simulink model "gnc_PathServer"  (R2026b)
settings: Solver=VariableStepAuto
values from neighbouring files (symbols this model uses):
  Ts = prm.Ts    [gnc_missionFSM.m]    (also in gnc_mpcPlantUpdate.m)
undefined symbols (not defined in the file or in its folder): P
libraries: drivinglib x3, simulink x2
settings Model: Creator=aomar  LastModifiedBy=aomar

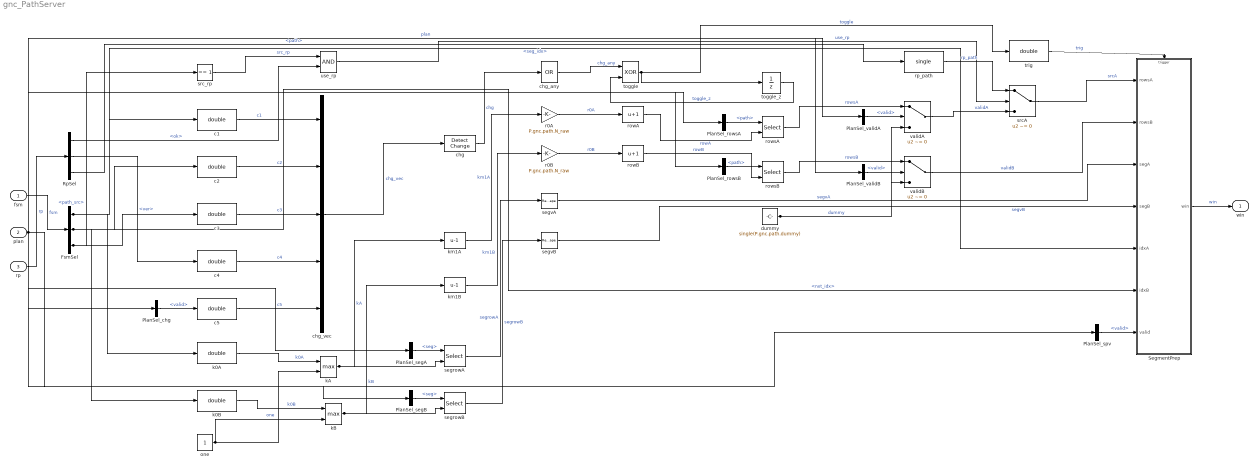
== system gnc_PathServer ==
  fsm : Inport  OutDataTypeStr=Bus: Bus_FsmOut  SampleTime=Ts.gnc
  plan : Inport  Port=2  OutDataTypeStr=Bus: Bus_MissionPlan
  rp : Inport  Port=3  OutDataTypeStr=Bus: Bus_ReplanResult  SampleTime=Ts.gnc
  FsmSel : BusSelector  OutputSignals=seg_idx,nxt_idx,path_src
  PlanSel_chg : BusSelector  OutputSignals=valid
  PlanSel_rowsA : BusSelector  OutputSignals=path
  PlanSel_rowsB : BusSelector  OutputSignals=path
  PlanSel_segA : BusSelector  OutputSignals=seg
  PlanSel_segB : BusSelector  OutputSignals=seg
  PlanSel_spv : BusSelector  OutputSignals=valid
  PlanSel_validA : BusSelector  OutputSignals=valid
  PlanSel_validB : BusSelector  OutputSignals=valid
  RpSel : BusSelector  OutputSignals=ok,ver,path
  SegmentPrep : Subsystem  TreatAsAtomicUnit=on
  c{1..5} (5 alike) : DataTypeConversion  OutDataTypeStr=double  RndMeth=Nearest
  chg : simulink/Logic and Bit Operations/Detect Change  vinit=0  OutDataTypeStr=boolean
  chg_any : Logic  Operator=OR  Inputs=1  AllPortsSameDT=off  OutDataTypeStr=boolean
  chg_vec : Concatenate  NumInputs=5
  dummy : Constant  Value=single(P.gnc.path.dummy)  OutDataTypeStr=single
  k0A : DataTypeConversion  OutDataTypeStr=double  RndMeth=Nearest
  k0B : DataTypeConversion  OutDataTypeStr=double  RndMeth=Nearest
  kA : MinMax  Function=max  Inputs=2
  kB : MinMax  Function=max  Inputs=2
  km1A : Bias  Bias=-1  SaturateOnIntegerOverflow=off
  km1B : Bias  Bias=-1  SaturateOnIntegerOverflow=off
  one : Constant  OutDataTypeStr=double  SampleTime=Ts.gnc
  r0A : Gain  Gain=P.gnc.path.N_raw
  r0B : Gain  Gain=P.gnc.path.N_raw
  rowA : Bias  Bias=1  SaturateOnIntegerOverflow=off
  rowB : Bias  Bias=1  SaturateOnIntegerOverflow=off
  rowsA : Selector  NumberOfDimensions=2  InputPortWidth=3  IndexOptions=Starting index (port),Select all  Indices=,  OutputSizes=P.gnc.path.N_raw,1
  rowsB : Selector  NumberOfDimensions=2  InputPortWidth=3  IndexOptions=Starting index (port),Select all  Indices=,  OutputSizes=P.gnc.path.N_raw,1
  rp_path : DataTypeConversion  OutDataTypeStr=single  RndMeth=Nearest
  segrowA : Selector  NumberOfDimensions=2  InputPortWidth=3  IndexOptions=Index vector (port),Select all  Indices=,  OutputSizes=1
  segrowB : Selector  NumberOfDimensions=2  InputPortWidth=3  IndexOptions=Index vector (port),Select all  Indices=,  OutputSizes=1
  segvA : Reshape
  segvB : Reshape
  srcA : Switch  Criteria=u2 ~= 0  SaturateOnIntegerOverflow=off  InputSameDT=off
  src_rp : simulink/Logic and Bit Operations/Compare To Constant  relop===  const=1  OutDataTypeStr=boolean
  toggle : Logic  Operator=XOR  AllPortsSameDT=off  OutDataTypeStr=boolean
  toggle_z : UnitDelay  InitialCondition=false  SampleTime=Ts.gnc
  trig : DataTypeConversion  OutDataTypeStr=double  RndMeth=Nearest
  use_rp : Logic  AllPortsSameDT=off  OutDataTypeStr=boolean
  validA : Switch  Criteria=u2 ~= 0  SaturateOnIntegerOverflow=off  InputSameDT=off
  validB : Switch  Criteria=u2 ~= 0  SaturateOnIntegerOverflow=off  InputSameDT=off
  win : Outport  OutDataTypeStr=Bus: Bus_PathWindow
  wires:
  fsm/1 -> FsmSel/1  "fsm"
  plan/1 -> PlanSel_segB/1, PlanSel_segA/1, PlanSel_validA/1, PlanSel_rowsA/1, PlanSel_spv/1, PlanSel_chg/1, PlanSel_rowsB/1, PlanSel_validB/1  "plan"
  rp/1 -> RpSel/1  "rp"
  RpSel/1 -> use_rp/2  "<ok>"
  RpSel/2 -> c4/1  "<ver>"
  RpSel/3 -> rp_path/1  "<path>"
  FsmSel/1 -> k0A/1, c1/1, SegmentPrep/5(idxA)  "<seg_idx>"
  FsmSel/2 -> k0B/1, c2/1, SegmentPrep/6(idxB)  "<nxt_idx>"
  FsmSel/3 -> src_rp/1, c3/1  "<path_src>"
  PlanSel_chg/1 -> c5/1  "<valid>"
  src_rp/1 -> use_rp/1  "src_rp"
  one/1 -> kA/2, kB/2  "one"
  c1/1 -> chg_vec/1  "c1"
  c2/1 -> chg_vec/2  "c2"
  c3/1 -> chg_vec/3  "c3"
  c4/1 -> chg_vec/4  "c4"
  c5/1 -> chg_vec/5  "c5"
  k0A/1 -> kA/1  "k0A"
  k0B/1 -> kB/1  "k0B"
  chg_vec/1 -> chg/1  "chg_vec"
  use_rp/1 -> srcA/2  "use_rp"
  kA/1 -> km1A/1, segrowA/2  "kA"
  kB/1 -> km1B/1, segrowB/2  "kB"
  PlanSel_segA/1 -> segrowA/1  "<seg>"
  PlanSel_segB/1 -> segrowB/1  "<seg>"
  km1A/1 -> r0A/1  "km1A"
  km1B/1 -> r0B/1  "km1B"
  segrowA/1 -> segvA/1  "segrowA"
  segrowB/1 -> segvB/1  "segrowB"
  chg/1 -> chg_any/1  "chg"
  chg_any/1 -> toggle/1  "chg_any"
  r0A/1 -> rowA/1  "r0A"
  r0B/1 -> rowB/1  "r0B"
  segvA/1 -> SegmentPrep/3(segA)  "segvA"
  segvB/1 -> SegmentPrep/4(segB)  "segvB"
  toggle/1 -> trig/1, toggle_z/1  "toggle"
  rowA/1 -> rowsA/2  "rowA"
  rowB/1 -> rowsB/2  "rowB"
  PlanSel_rowsA/1 -> rowsA/1  "<path>"
  PlanSel_rowsB/1 -> rowsB/1  "<path>"
  dummy/1 -> validA/3, validB/3  "dummy"
  toggle_z/1 -> toggle/2  "toggle_z"
  rowsA/1 -> validA/1  "rowsA"
  rowsB/1 -> validB/1  "rowsB"
  PlanSel_validA/1 -> validA/2  "<valid>"
  PlanSel_validB/1 -> validB/2  "<valid>"
  validA/1 -> srcA/3  "validA"
  validB/1 -> SegmentPrep/2(rowsB)  "validB"
  rp_path/1 -> srcA/1  "rp_path"
  srcA/1 -> SegmentPrep/1(rowsA)  "srcA"
  trig/1 -> SegmentPrep/Trigger  "trig"
  PlanSel_spv/1 -> SegmentPrep/7(valid)  "<valid>"
  SegmentPrep/1(win) -> win/1  "win"

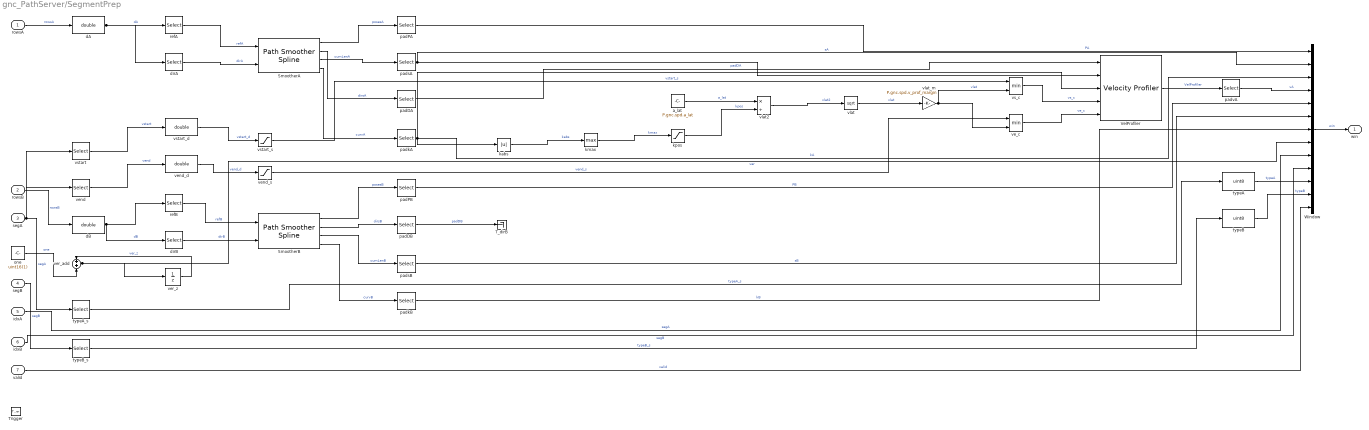
== system gnc_PathServer/SegmentPrep ==
  rowsA : Inport
  rowsB : Inport  Port=2
  segA : Inport  Port=3
  segB : Inport  Port=4
  idxA : Inport  Port=5
  idxB : Inport  Port=6
  valid : Inport  Port=7
  Trigger : TriggerPort  TriggerType=either  VariantControl=(inherit)  InitialTriggerSignalState=zero  PortDimensions=1
  SmootherA : drivinglib/Path Smoother Spline  NumSmoothPoses=P.gnc.path.N_smooth  MinSeparation=1e-3  SampleTime=-1  ShowOptionalOutports=on  SimulateUsing=Code generation
  SmootherB : drivinglib/Path Smoother Spline  NumSmoothPoses=P.gnc.path.N_smooth  MinSeparation=1e-3  SampleTime=-1  ShowOptionalOutports=on  SimulateUsing=Code generation
  T_dirB : Terminator
  VelProfiler : drivinglib/Velocity Profiler  MaxLongitudinalAccel=P.gnc.spd.a_acc  MaxLongitudinalDecel=P.gnc.spd.a_dec  MaxSpeed=P.gnc.spd.v_max  MaxLongitudinalJerk=P.gnc.spd.jerk  MaxLateralAccel=P.gnc.spd.a_lat  ShowOptionalOutport=off  SampleTime=-1  SimulateUsing=Code generation
  Window : BusCreator  Inputs=13  OutDataTypeStr=Bus: Bus_PathWindow  NonVirtualBus=on
  a_lat : Constant  Value=P.gnc.spd.a_lat  OutDataTypeStr=double  SampleTime=-1
  dA : DataTypeConversion  OutDataTypeStr=double  RndMeth=Nearest
  dB : DataTypeConversion  OutDataTypeStr=double  RndMeth=Nearest
  dirA : Selector  NumberOfDimensions=2  InputPortWidth=3  IndexOptions=Select all,Index vector (dialog)  Indices=,4  OutputSizes=1
  dirB : Selector  NumberOfDimensions=2  InputPortWidth=3  IndexOptions=Select all,Index vector (dialog)  Indices=,4  OutputSizes=1
  kabs : Abs  SaturateOnIntegerOverflow=off
  kmax : MinMax  Function=max
  kpos : Saturate  UpperLimit=inf  LowerLimit=1e-9
  one : Constant  Value=uint16(1)  OutDataTypeStr=uint16  SampleTime=-1
  padDA : Selector  IndexOptions=Index vector (dialog)  Indices=1:P.gnc.path.N_smooth  OutputSizes=1
  padDB : Selector  IndexOptions=Index vector (dialog)  Indices=1:P.gnc.path.N_smooth  OutputSizes=1
  padPA : Selector  NumberOfDimensions=2  InputPortWidth=3  IndexOptions=Index vector (dialog),Index vector (dialog)  Indices=1:P.gnc.path.N_smooth,[1 2 3]  OutputSizes=1
  padPB : Selector  NumberOfDimensions=2  InputPortWidth=3  IndexOptions=Index vector (dialog),Index vector (dialog)  Indices=1:P.gnc.path.N_smooth,[1 2 3]  OutputSizes=1
  padkA : Selector  IndexOptions=Index vector (dialog)  Indices=1:P.gnc.path.N_smooth  OutputSizes=1
  padkB : Selector  IndexOptions=Index vector (dialog)  Indices=1:P.gnc.path.N_smooth  OutputSizes=1
  padsA : Selector  IndexOptions=Index vector (dialog)  Indices=1:P.gnc.path.N_smooth  OutputSizes=1
  padsB : Selector  IndexOptions=Index vector (dialog)  Indices=1:P.gnc.path.N_smooth  OutputSizes=1
  padvA : Selector  IndexOptions=Index vector (dialog)  Indices=1:P.gnc.path.N_smooth  OutputSizes=1
  refA : Selector  NumberOfDimensions=2  InputPortWidth=3  IndexOptions=Select all,Index vector (dialog)  Indices=,[1 2 3]  OutputSizes=1
  refB : Selector  NumberOfDimensions=2  InputPortWidth=3  IndexOptions=Select all,Index vector (dialog)  Indices=,[1 2 3]  OutputSizes=1
  typeA : DataTypeConversion  OutDataTypeStr=uint8  RndMeth=Nearest
  typeA_s : Selector  IndexOptions=Index vector (dialog)  Indices=1  OutputSizes=1
  typeB : DataTypeConversion  OutDataTypeStr=uint8  RndMeth=Nearest
  typeB_s : Selector  IndexOptions=Index vector (dialog)  Indices=1  OutputSizes=1
  ve_c : MinMax  Inputs=2
  vend : Selector  IndexOptions=Index vector (dialog)  Indices=5  OutputSizes=1
  vend_d : DataTypeConversion  OutDataTypeStr=double  RndMeth=Nearest
  vend_s : Saturate  UpperLimit=P.gnc.spd.v_max  LowerLimit=0
  ver_add : Sum  OutDataTypeStr=uint16
  ver_z : UnitDelay  InitialCondition=uint16(0)  SampleTime=-1
  vlat : Sqrt
  vlat2 : Product  Inputs=*/
  vlat_m : Gain  Gain=P.gnc.spd.v_prof_margin
  vs_c : MinMax  Inputs=2
  vstart : Selector  IndexOptions=Index vector (dialog)  Indices=4  OutputSizes=1
  vstart_d : DataTypeConversion  OutDataTypeStr=double  RndMeth=Nearest
  vstart_s : Saturate  UpperLimit=P.gnc.spd.v_max  LowerLimit=0
  win : Outport  OutDataTypeStr=Bus: Bus_PathWindow  InitialOutput=P.ic.Bus_PathWindow
  wires:
  rowsA/1 -> dA/1  "rowsA"
  rowsB/1 -> dB/1  "rowsB"
  segA/1 -> typeA_s/1, vstart/1, vend/1  "segA"
  one/1 -> ver_add/2  "one"
  segB/1 -> typeB_s/1  "segB"
  idxA/1 -> Window/9  "segA"
  idxB/1 -> Window/10  "segB"
  valid/1 -> Window/13  "valid"
  ver_add/1 -> Window/8, ver_z/1  "ver"
  vstart/1 -> vstart_d/1  "vstart"
  vend/1 -> vend_d/1  "vend"
  typeA_s/1 -> typeA/1  "typeA_s"
  typeB_s/1 -> typeB/1  "typeB_s"
  dA/1 -> dirA/1, refA/1  "dA"
  dB/1 -> refB/1, dirB/1  "dB"
  ver_z/1 -> ver_add/1  "ver_z"
  refA/1 -> SmootherA/1  "refA"
  dirA/1 -> SmootherA/2  "dirA"
  refB/1 -> SmootherB/1  "refB"
  dirB/1 -> SmootherB/2  "dirB"
  vstart_d/1 -> vstart_s/1  "vstart_d"
  vend_d/1 -> vend_s/1  "vend_d"
  vstart_s/1 -> vs_c/1  "vstart_s"
  vend_s/1 -> ve_c/1  "vend_s"
  SmootherA/1 -> padPA/1  "posesA"
  SmootherA/2 -> padDA/1  "dirsA"
  SmootherA/3 -> padsA/1  "cumLenA"
  SmootherA/4 -> padkA/1  "curvA"
  SmootherB/1 -> padPB/1  "posesB"
  SmootherB/2 -> padDB/1  "dirsB"
  SmootherB/3 -> padsB/1  "cumLenB"
  SmootherB/4 -> padkB/1  "curvB"
  padPA/1 -> Window/1  "PA"
  padsA/1 -> VelProfiler/2, Window/2  "sA"
  padDA/1 -> VelProfiler/1  "padDA"
  padkA/1 -> Window/3, VelProfiler/3, kabs/1  "kA"
  padPB/1 -> Window/5  "PB"
  padDB/1 -> T_dirB/1  "padDB"
  padsB/1 -> Window/6  "sB"
  padkB/1 -> Window/7  "kB"
  kabs/1 -> kmax/1  "kabs"
  kmax/1 -> kpos/1  "kmax"
  a_lat/1 -> vlat2/1  "a_lat"
  kpos/1 -> vlat2/2  "kpos"
  vlat2/1 -> vlat/1  "vlat2"
  vlat/1 -> vlat_m/1  "vlat"
  vlat_m/1 -> ve_c/2, vs_c/2  "vlat"
  vs_c/1 -> VelProfiler/4  "vs_c"
  ve_c/1 -> VelProfiler/5  "ve_c"
  VelProfiler/1 -> padvA/1  "VelProfiler"
  padvA/1 -> Window/4  "vA"
  typeA/1 -> Window/11  "typeA"
  typeB/1 -> Window/12  "typeB"
  Window/1 -> win/1  "win"
